simulink model "gofa_robot"  (R2023a)
settings: Solver=FixedStepAuto  StartTime=0.0  StopTime=11  FixedStep=0.001  RelTol=1e-3
undefined symbols (not defined in the file or in its folder): X, Y, Z
libraries: sm_lib x58, nesl_utility x10, slpidlib x3
(part 6 of 7)

== matlab function gofa_robot/gofa_FK2 ==
  data: x output; q1 input; y output; q2 input; q3 input; q4 input; q5 input; q6 input; z output; R output
function [x,y,z,R] = fcn(q1,q2,q3,q4,q5,q6)

R=zeros(3,3);

R(1,1)= (24678615572571482867467662723121*cos(q6)*(cos(q5)*(cos(q3)*(cos(q1)*sin(q2 + pi/2) + (4967757600021511*cos(q2 + pi/2)*sin(q1))/81129638414606681695789005144064) - (4967757600021511*sin(q1))/81129638414606681695789005144064 + sin(q3)*(cos(q1)*cos(q2 + pi/2) - (4967757600021511*sin(q1)*sin(q2 + pi/2))/81129638414606681695789005144064)) + (4967757600021511*cos(q5)*(cos(q4)*sin(q1) + (4967757600021511*cos(q4)*(cos(q3)*(cos(q1)*sin(q2 + pi/2) + (4967757600021511*cos(q2 + pi/2)*sin(q1))/81129638414606681695789005144064) + sin(q3)*(cos(q1)*cos(q2 + pi/2) - (4967757600021511*sin(q1)*sin(q2 + pi/2))/81129638414606681695789005144064)))/81129638414606681695789005144064 + sin(q4)*(cos(q3)*(cos(q1)*cos(q2 + pi/2) - (4967757600021511*sin(q1)*sin(q2 + pi/2))/81129638414606681695789005144064) - sin(q3)*(cos(q1)*sin(q2 + pi/2) + (4967757600021511*cos(q2 + pi/2)*sin(q1))/81129638414606681695789005144064))))/81129638414606681695789005144064 - sin(q5)*(sin(q1)*sin(q4) - cos(q4)*(cos(q3)*(cos(q1)*cos(q2 + pi/2) - (4967757600021511*sin(q1)*sin(q2 + pi/2))/81129638414606681695789005144064) - sin(q3)*(cos(q1)*sin(q2 + pi/2) + (4967757600021511*cos(q2 + pi/2)*sin(q1))/81129638414606681695789005144064)) + (4967757600021511*sin(q4)*(cos(q3)*(cos(q1)*sin(q2 + pi/2) + (4967757600021511*cos(q2 + pi/2)*sin(q1))/81129638414606681695789005144064) + sin(q3)*(cos(q1)*cos(q2 + pi/2) - (4967757600021511*sin(q1)*sin(q2 + pi/2))/81129638414606681695789005144064)))/81129638414606681695789005144064)))/3291009114642412084309938365114701009965471731267159726697218048 - cos(q6)*(sin(q5)*(cos(q3)*(cos(q1)*sin(q2 + pi/2) + (4967757600021511*cos(q2 + pi/2)*sin(q1))/81129638414606681695789005144064) - (4967757600021511*sin(q1))/81129638414606681695789005144064 + sin(q3)*(cos(q1)*cos(q2 + pi/2) - (4967757600021511*sin(q1)*sin(q2 + pi/2))/81129638414606681695789005144064)) + (4967757600021511*sin(q5)*(cos(q4)*sin(q1) + (4967757600021511*cos(q4)*(cos(q3)*(cos(q1)*sin(q2 + pi/2) + (4967757600021511*cos(q2 + pi/2)*sin(q1))/81129638414606681695789005144064) + sin(q3)*(cos(q1)*cos(q2 + pi/2) - (4967757600021511*sin(q1)*sin(q2 + pi/2))/81129638414606681695789005144064)))/81129638414606681695789005144064 + sin(q4)*(cos(q3)*(cos(q1)*cos(q2 + pi/2) - (4967757600021511*sin(q1)*sin(q2 + pi/2))/81129638414606681695789005144064) - sin(q3)*(cos(q1)*sin(q2 + pi/2) + (4967757600021511*cos(q2 + pi/2)*sin(q1))/81129638414606681695789005144064))))/81129638414606681695789005144064 + cos(q5)*(sin(q1)*sin(q4) - cos(q4)*(cos(q3)*(cos(q1)*cos(q2 + pi/2) - (4967757600021511*sin(q1)*sin(q2 + pi/2))/81129638414606681695789005144064) - sin(q3)*(cos(q1)*sin(q2 + pi/2) + (4967757600021511*cos(q2 + pi/2)*sin(q1))/81129638414606681695789005144064)) + (4967757600021511*sin(q4)*(cos(q3)*(cos(q1)*sin(q2 + pi/2) + (4967757600021511*cos(q2 + pi/2)*sin(q1))/81129638414606681695789005144064) + sin(q3)*(cos(q1)*cos(q2 + pi/2) - (4967757600021511*sin(q1)*sin(q2 + pi/2))/81129638414606681695789005144064)))/81129638414606681695789005144064)) - (4967757600021511*sin(q6)*(cos(q5)*(cos(q3)*(cos(q1)*sin(q2 + pi/2) + (4967757600021511*cos(q2 + pi/2)*sin(q1))/81129638414606681695789005144064) - (4967757600021511*sin(q1))/81129638414606681695789005144064 + sin(q3)*(cos(q1)*cos(q2 + pi/2) - (4967757600021511*sin(q1)*sin(q2 + pi/2))/81129638414606681695789005144064)) + (4967757600021511*cos(q5)*(cos(q4)*sin(q1) + (4967757600021511*cos(q4)*(cos(q3)*(cos(q1)*sin(q2 + pi/2) + (4967757600021511*cos(q2 + pi/2)*sin(q1))/81129638414606681695789005144064) + sin(q3)*(cos(q1)*cos(q2 + pi/2) - (4967757600021511*sin(q1)*sin(q2 + pi/2))/81129638414606681695789005144064)))/81129638414606681695789005144064 + sin(q4)*(cos(q3)*(cos(q1)*cos(q2 + pi/2) - (4967757600021511*sin(q1)*sin(q2 + pi/2))/81129638414606681695789005144064) - sin(q3)*(cos(q1)*sin(q2 + pi/2) + (4967757600021511*cos(q2 + pi/2)*sin(q1))/81129638414606681695789005144064))))/81129638414606681695789005144064 - sin(q5)*(sin(q1)*sin(q4) - cos(q4)*(cos(q3)*(cos(q1)*cos(q2 + pi/2) - (4967757600021511*sin(q1)*sin(q2 + pi/2))/81129638414606681695789005144064) - sin(q3)*(cos(q1)*sin(q2 + pi/2) + (4967757600021511*cos(q2 + pi/2)*sin(q1))/81129638414606681695789005144064)) + (4967757600021511*sin(q4)*(cos(q3)*(cos(q1)*sin(q2 + pi/2) + (4967757600021511*cos(q2 + pi/2)*sin(q1))/81129638414606681695789005144064) + sin(q3)*(cos(q1)*cos(q2 + pi/2) - (4967757600021511*sin(q1)*sin(q2 + pi/2))/81129638414606681695789005144064)))/81129638414606681695789005144064)))/81129638414606681695789005144064 - (4967757600021511*sin(q6)*(sin(q5)*(cos(q3)*(cos(q1)*sin(q2 + pi/2) + (4967757600021511*cos(q2 + pi/2)*sin(q1))/81129638414606681695789005144064) - (4967757600021511*sin(q1))/81129638414606681695789005144064 + sin(q3)*(cos(q1)*cos(q2 + pi/2) - (4967757600021511*sin(q1)*sin(q2 + pi/2))/81129638414606681695789005144064)) + (4967757600021511*sin(q5)*(cos(q4)*sin(q1) + (4967757600021511*cos(q4)*(cos(q3)*(cos(q1)*sin(q2 + pi/2) + (4967757600021511*cos(q2 + pi/2)*sin(q1))/81129638414606681695789005144064) + sin(q3)*(cos(q1)*cos(q2 + pi/2) - (4967757600021511*sin(q1)*sin(q2 + pi/2))/81129638414606681695789005144064)))/81129638414606681695789005144064 + sin(q4)*(cos(q3)*(cos(q1)*cos(q2 + pi/2) - (4967757600021511*sin(q1)*sin(q2 + pi/2))/81129638414606681695789005144064) - sin(q3)*(cos(q1)*sin(q2 + pi/2) + (4967757600021511*cos(q2 + pi/2)*sin(q1))/81129638414606681695789005144064))))/81129638414606681695789005144064 + cos(q5)*(sin(q1)*sin(q4) - cos(q4)*(cos(q3)*(cos(q1)*cos(q2 + pi/2) - (4967757600021511*sin(q1)*sin(q2 + pi/2))/81129638414606681695789005144064) - sin(q3)*(cos(q1)*sin(q2 + pi/2) + (4967757600021511*cos(q2 + pi/2)*sin(q1))/81129638414606681695789005144064)) + (4967757600021511*sin(q4)*(cos(q3)*(cos(q1)*sin(q2 + pi/2) + (4967757600021511*cos(q2 + pi/2)*sin(q1))/81129638414606681695789005144064) + sin(q3)*(cos(q1)*cos(q2 + pi/2) - (4967757600021511*sin(q1)*sin(q2 + pi/2))/81129638414606681695789005144064)))/81129638414606681695789005144064)))/40564819207303340847894502572032 + (4967757600021511*cos(q6)*((24678615572571482867467662723121*sin(q1))/6582018229284824168619876730229402019930943462534319453394436096 - (4967757600021511*cos(q3)*(cos(q1)*sin(q2 + pi/2) + (4967757600021511*cos(q2 + pi/2)*sin(q1))/81129638414606681695789005144064))/81129638414606681695789005144064 + cos(q4)*sin(q1) - (4967757600021511*sin(q3)*(cos(q1)*cos(q2 + pi/2) - (4967757600021511*sin(q1)*sin(q2 + pi/2))/81129638414606681695789005144064))/81129638414606681695789005144064 + (4967757600021511*cos(q4)*(cos(q3)*(cos(q1)*sin(q2 + pi/2) + (4967757600021511*cos(q2 + pi/2)*sin(q1))/81129638414606681695789005144064) + sin(q3)*(cos(q1)*cos(q2 + pi/2) - (4967757600021511*sin(q1)*sin(q2 + pi/2))/81129638414606681695789005144064)))/81129638414606681695789005144064 + sin(q4)*(cos(q3)*(cos(q1)*cos(q2 + pi/2) - (4967757600021511*sin(q1)*sin(q2 + pi/2))/81129638414606681695789005144064) - sin(q3)*(cos(q1)*sin(q2 + pi/2) + (4967757600021511*cos(q2 + pi/2)*sin(q1))/81129638414606681695789005144064))))/40564819207303340847894502572032 - sin(q6)*((24678615572571482867467662723121*sin(q1))/6582018229284824168619876730229402019930943462534319453394436096 - (4967757600021511*cos(q3)*(cos(q1)*sin(q2 + pi/2) + (4967757600021511*cos(q2 + pi/2)*sin(q1))/81129638414606681695789005144064))/81129638414606681695789005144064 + cos(q4)*sin(q1) - (4967757600021511*sin(q3)*(cos(q1)*cos(q2 + pi/2) - (4967757600021511*sin(q1)*sin(q2 + pi/2))/81129638414606681695789005144064))/81129638414606681695789005144064 + (4967757600021511*cos(q4)*(cos(q3)*(cos(q1)*sin(q2 + pi/2) + (4967757600021511*cos(q2 + pi/2)*sin(q1))/81129638414606681695789005144064) + sin(q3)*(cos(q1)*cos(q2 + pi/2) - (4967757600021511*sin(q1)*sin(q2 + pi/2))/81129638414606681695789005144064)))/81129638414606681695789005144064 + sin(q4)*(cos(q3)*(cos(q1)*cos(q2 + pi/2) - (4967757600021511*sin(q1)*sin(q2 + pi/2))/81129638414606681695789005144064) - sin(q3)*(cos(q1)*sin(q2 + pi/2) + (4967757600021511*cos(q2 + pi/2)*sin(q1))/81129638414606681695789005144064)));
R(1,2)= sin(q6)*(sin(q5)*(cos(q3)*(cos(q1)*sin(q2 + pi/2) + (4967757600021511*cos(q2 + pi/2)*sin(q1))/81129638414606681695789005144064) - (4967757600021511*sin(q1))/81129638414606681695789005144064 + sin(q3)*(cos(q1)*cos(q2 + pi/2) - (4967757600021511*sin(q1)*sin(q2 + pi/2))/81129638414606681695789005144064)) + (4967757600021511*sin(q5)*(cos(q4)*sin(q1) + (4967757600021511*cos(q4)*(cos(q3)*(cos(q1)*sin(q2 + pi/2) + (4967757600021511*cos(q2 + pi/2)*sin(q1))/81129638414606681695789005144064) + sin(q3)*(cos(q1)*cos(q2 + pi/2) - (4967757600021511*sin(q1)*sin(q2 + pi/2))/81129638414606681695789005144064)))/81129638414606681695789005144064 + sin(q4)*(cos(q3)*(cos(q1)*cos(q2 + pi/2) - (4967757600021511*sin(q1)*sin(q2 + pi/2))/81129638414606681695789005144064) - sin(q3)*(cos(q1)*sin(q2 + pi/2) + (4967757600021511*cos(q2 + pi/2)*sin(q1))/81129638414606681695789005144064))))/81129638414606681695789005144064 + cos(q5)*(sin(q1)*sin(q4) - cos(q4)*(cos(q3)*(cos(q1)*cos(q2 + pi/2) - (4967757600021511*sin(q1)*sin(q2 + pi/2))/81129638414606681695789005144064) - sin(q3)*(cos(q1)*sin(q2 + pi/2) + (4967757600021511*cos(q2 + pi/2)*sin(q1))/81129638414606681695789005144064)) + (4967757600021511*sin(q4)*(cos(q3)*(cos(q1)*sin(q2 + pi/2) + (4967757600021511*cos(q2 + pi/2)*sin(q1))/81129638414606681695789005144064) + sin(q3)*(cos(q1)*cos(q2 + pi/2) - (4967757600021511*sin(q1)*sin(q2 + pi/2))/81129638414606681695789005144064)))/81129638414606681695789005144064)) - (4967757600021511*cos(q6)*(sin(q5)*(cos(q3)*(cos(q1)*sin(q2 + pi/2) + (4967757600021511*cos(q2 + pi/2)*sin(q1))/81129638414606681695789005144064) - (4967757600021511*sin(q1))/81129638414606681695789005144064 + sin(q3)*(cos(q1)*cos(q2 + pi/2) - (4967757600021511*sin(q1)*sin(q2 + pi/2))/81129638414606681695789005144064)) + (4967757600021511*sin(q5)*(cos(q4)*sin(q1) + (4967757600021511*cos(q4)*(cos(q3)*(cos(q1)*sin(q2 + pi/2) + (4967757600021511*cos(q2 + pi/2)*sin(q1))/81129638414606681695789005144064) + sin(q3)*(cos(q1)*cos(q2 + pi/2) - (4967757600021511*sin(q1)*sin(q2 + pi/2))/81129638414606681695789005144064)))/81129638414606681695789005144064 + sin(q4)*(cos(q3)*(cos(q1)*cos(q2 + pi/2) - (4967757600021511*sin(q1)*sin(q2 + pi/2))/81129638414606681695789005144064) - sin(q3)*(cos(q1)*sin(q2 + pi/2) + (4967757600021511*cos(q2 + pi/2)*sin(q1))/81129638414606681695789005144064))))/81129638414606681695789005144064 + cos(q5)*(sin(q1)*sin(q4) - cos(q4)*(cos(q3)*(cos(q1)*cos(q2 + pi/2) - (4967757600021511*sin(q1)*sin(q2 + pi/2))/81129638414606681695789005144064) - sin(q3)*(cos(q1)*sin(q2 + pi/2) + (4967757600021511*cos(q2 + pi/2)*sin(q1))/81129638414606681695789005144064)) + (4967757600021511*sin(q4)*(cos(q3)*(cos(q1)*sin(q2 + pi/2) + (4967757600021511*cos(q2 + pi/2)*sin(q1))/81129638414606681695789005144064) + sin(q3)*(cos(q1)*cos(q2 + pi/2) - (4967757600021511*sin(q1)*sin(q2 + pi/2))/81129638414606681695789005144064)))/81129638414606681695789005144064)))/40564819207303340847894502572032 - (24678615572571482867467662723121*sin(q6)*(cos(q5)*(cos(q3)*(cos(q1)*sin(q2 + pi/2) + (4967757600021511*cos(q2 + pi/2)*sin(q1))/81129638414606681695789005144064) - (4967757600021511*sin(q1))/81129638414606681695789005144064 + sin(q3)*(cos(q1)*cos(q2 + pi/2) - (4967757600021511*sin(q1)*sin(q2 + pi/2))/81129638414606681695789005144064)) + (4967757600021511*cos(q5)*(cos(q4)*sin(q1) + (4967757600021511*cos(q4)*(cos(q3)*(cos(q1)*sin(q2 + pi/2) + (4967757600021511*cos(q2 + pi/2)*sin(q1))/81129638414606681695789005144064) + sin(q3)*(cos(q1)*cos(q2 + pi/2) - (4967757600021511*sin(q1)*sin(q2 + pi/2))/81129638414606681695789005144064)))/81129638414606681695789005144064 + sin(q4)*(cos(q3)*(cos(q1)*cos(q2 + pi/2) - (4967757600021511*sin(q1)*sin(q2 + pi/2))/81129638414606681695789005144064) - sin(q3)*(cos(q1)*sin(q2 + pi/2) + (4967757600021511*cos(q2 + pi/2)*sin(q1))/81129638414606681695789005144064))))/81129638414606681695789005144064 - sin(q5)*(sin(q1)*sin(q4) - cos(q4)*(cos(q3)*(cos(q1)*cos(q2 + pi/2) - (4967757600021511*sin(q1)*sin(q2 + pi/2))/81129638414606681695789005144064) - sin(q3)*(cos(q1)*sin(q2 + pi/2) + (4967757600021511*cos(q2 + pi/2)*sin(q1))/81129638414606681695789005144064)) + (4967757600021511*sin(q4)*(cos(q3)*(cos(q1)*sin(q2 + pi/2) + (4967757600021511*cos(q2 + pi/2)*sin(q1))/81129638414606681695789005144064) + sin(q3)*(cos(q1)*cos(q2 + pi/2) - (4967757600021511*sin(q1)*sin(q2 + pi/2))/81129638414606681695789005144064)))/81129638414606681695789005144064)))/3291009114642412084309938365114701009965471731267159726697218048 - (4967757600021511*cos(q6)*(cos(q5)*(cos(q3)*(cos(q1)*sin(q2 + pi/2) + (4967757600021511*cos(q2 + pi/2)*sin(q1))/81129638414606681695789005144064) - (4967757600021511*sin(q1))/81129638414606681695789005144064 + sin(q3)*(cos(q1)*cos(q2 + pi/2) - (4967757600021511*sin(q1)*sin(q2 + pi/2))/81129638414606681695789005144064)) + (4967757600021511*cos(q5)*(cos(q4)*sin(q1) + (4967757600021511*cos(q4)*(cos(q3)*(cos(q1)*sin(q2 + pi/2) + (4967757600021511*cos(q2 + pi/2)*sin(q1))/81129638414606681695789005144064) + sin(q3)*(cos(q1)*cos(q2 + pi/2) - (4967757600021511*sin(q1)*sin(q2 + pi/2))/81129638414606681695789005144064)))/81129638414606681695789005144064 + sin(q4)*(cos(q3)*(cos(q1)*cos(q2 + pi/2) - (4967757600021511*sin(q1)*sin(q2 + pi/2))/81129638414606681695789005144064) - sin(q3)*(cos(q1)*sin(q2 + pi/2) + (4967757600021511*cos(q2 + pi/2)*sin(q1))/81129638414606681695789005144064))))/81129638414606681695789005144064 - sin(q5)*(sin(q1)*sin(q4) - cos(q4)*(cos(q3)*(cos(q1)*cos(q2 + pi/2) - (4967757600021511*sin(q1)*sin(q2 + pi/2))/81129638414606681695789005144064) - sin(q3)*(cos(q1)*sin(q2 + pi/2) + (4967757600021511*cos(q2 + pi/2)*sin(q1))/81129638414606681695789005144064)) + (4967757600021511*sin(q4)*(cos(q3)*(cos(q1)*sin(q2 + pi/2) + (4967757600021511*cos(q2 + pi/2)*sin(q1))/81129638414606681695789005144064) + sin(q3)*(cos(q1)*cos(q2 + pi/2) - (4967757600021511*sin(q1)*sin(q2 + pi/2))/81129638414606681695789005144064)))/81129638414606681695789005144064)))/81129638414606681695789005144064 - cos(q6)*((24678615572571482867467662723121*sin(q1))/6582018229284824168619876730229402019930943462534319453394436096 - (4967757600021511*cos(q3)*(cos(q1)*sin(q2 + pi/2) + (4967757600021511*cos(q2 + pi/2)*sin(q1))/81129638414606681695789005144064))/81129638414606681695789005144064 + cos(q4)*sin(q1) - (4967757600021511*sin(q3)*(cos(q1)*cos(q2 + pi/2) - (4967757600021511*sin(q1)*sin(q2 + pi/2))/81129638414606681695789005144064))/81129638414606681695789005144064 + (4967757600021511*cos(q4)*(cos(q3)*(cos(q1)*sin(q2 + pi/2) + (4967757600021511*cos(q2 + pi/2)*sin(q1))/81129638414606681695789005144064) + sin(q3)*(cos(q1)*cos(q2 + pi/2) - (4967757600021511*sin(q1)*sin(q2 + pi/2))/81129638414606681695789005144064)))/81129638414606681695789005144064 + sin(q4)*(cos(q3)*(cos(q1)*cos(q2 + pi/2) - (4967757600021511*sin(q1)*sin(q2 + pi/2))/81129638414606681695789005144064) - sin(q3)*(cos(q1)*sin(q2 + pi/2) + (4967757600021511*cos(q2 + pi/2)*sin(q1))/81129638414606681695789005144064))) - (4967757600021511*sin(q6)*((24678615572571482867467662723121*sin(q1))/6582018229284824168619876730229402019930943462534319453394436096 - (4967757600021511*cos(q3)*(cos(q1)*sin(q2 + pi/2) + (4967757600021511*cos(q2 + pi/2)*sin(q1))/81129638414606681695789005144064))/81129638414606681695789005144064 + cos(q4)*sin(q1) - (4967757600021511*sin(q3)*(cos(q1)*cos(q2 + pi/2) - (4967757600021511*sin(q1)*sin(q2 + pi/2))/81129638414606681695789005144064))/81129638414606681695789005144064 + (4967757600021511*cos(q4)*(cos(q3)*(cos(q1)*sin(q2 + pi/2) + (4967757600021511*cos(q2 + pi/2)*sin(q1))/81129638414606681695789005144064) + sin(q3)*(cos(q1)*cos(q2 + pi/2) - (4967757600021511*sin(q1)*sin(q2 + pi/2))/81129638414606681695789005144064)))/81129638414606681695789005144064 + sin(q4)*(cos(q3)*(cos(q1)*cos(q2 + pi/2) - (4967757600021511*sin(q1)*sin(q2 + pi/2))/81129638414606681695789005144064) - sin(q3)*(cos(q1)*sin(q2 + pi/2) + (4967757600021511*cos(q2 + pi/2)*sin(q1))/81129638414606681695789005144064))))/40564819207303340847894502572032; 
R(1,3)= (24678615572571482867467662723121*cos(q3)*(cos(q1)*sin(q2 + pi/2) + (4967757600021511*cos(q2 + pi/2)*sin(q1))/81129638414606681695789005144064))/6582018229284824168619876730229402019930943462534319453394436096 - (122597380068651197257713859414983140362437055831*sin(q1))/533996758980227520598755426542388028650676130589163192486760401955554931445160137505740521734144 - (4967757600021511*cos(q4)*sin(q1))/81129638414606681695789005144064 + (24678615572571482867467662723121*sin(q3)*(cos(q1)*cos(q2 + pi/2) - (4967757600021511*sin(q1)*sin(q2 + pi/2))/81129638414606681695789005144064))/6582018229284824168619876730229402019930943462534319453394436096 + cos(q5)*(cos(q3)*(cos(q1)*sin(q2 + pi/2) + (4967757600021511*cos(q2 + pi/2)*sin(q1))/81129638414606681695789005144064) - (4967757600021511*sin(q1))/81129638414606681695789005144064 + sin(q3)*(cos(q1)*cos(q2 + pi/2) - (4967757600021511*sin(q1)*sin(q2 + pi/2))/81129638414606681695789005144064)) + (4967757600021511*cos(q5)*(cos(q4)*sin(q1) + (4967757600021511*cos(q4)*(cos(q3)*(cos(q1)*sin(q2 + pi/2) + (4967757600021511*cos(q2 + pi/2)*sin(q1))/81129638414606681695789005144064) + sin(q3)*(cos(q1)*cos(q2 + pi/2) - (4967757600021511*sin(q1)*sin(q2 + pi/2))/81129638414606681695789005144064)))/81129638414606681695789005144064 + sin(q4)*(cos(q3)*(cos(q1)*cos(q2 + pi/2) - (4967757600021511*sin(q1)*sin(q2 + pi/2))/81129638414606681695789005144064) - sin(q3)*(cos(q1)*sin(q2 + pi/2) + (4967757600021511*cos(q2 + pi/2)*sin(q1))/81129638414606681695789005144064))))/81129638414606681695789005144064 - sin(q5)*(sin(q1)*sin(q4) - cos(q4)*(cos(q3)*(cos(q1)*cos(q2 + pi/2) - (4967757600021511*sin(q1)*sin(q2 + pi/2))/81129638414606681695789005144064) - sin(q3)*(cos(q1)*sin(q2 + pi/2) + (4967757600021511*cos(q2 + pi/2)*sin(q1))/81129638414606681695789005144064)) + (4967757600021511*sin(q4)*(cos(q3)*(cos(q1)*sin(q2 + pi/2) + (4967757600021511*cos(q2 + pi/2)*sin(q1))/81129638414606681695789005144064) + sin(q3)*(cos(q1)*cos(q2 + pi/2) - (4967757600021511*sin(q1)*sin(q2 + pi/2))/81129638414606681695789005144064)))/81129638414606681695789005144064) - (24678615572571482867467662723121*cos(q4)*(cos(q3)*(cos(q1)*sin(q2 + pi/2) + (4967757600021511*cos(q2 + pi/2)*sin(q1))/81129638414606681695789005144064) + sin(q3)*(cos(q1)*cos(q2 + pi/2) - (4967757600021511*sin(q1)*sin(q2 + pi/2))/81129638414606681695789005144064)))/6582018229284824168619876730229402019930943462534319453394436096 - (4967757600021511*sin(q4)*(cos(q3)*(cos(q1)*cos(q2 + pi/2) - (4967757600021511*sin(q1)*sin(q2 + pi/2))/81129638414606681695789005144064) - sin(q3)*(cos(q1)*sin(q2 + pi/2) + (4967757600021511*cos(q2 + pi/2)*sin(q1))/81129638414606681695789005144064)))/81129638414606681695789005144064;
R(2,1)= (24678615572571482867467662723121*cos(q6)*(cos(q5)*((4967757600021511*cos(q1))/81129638414606681695789005144064 - cos(q3)*((4967757600021511*cos(q1)*cos(q2 + pi/2))/81129638414606681695789005144064 - sin(q1)*sin(q2 + pi/2)) + sin(q3)*((4967757600021511*cos(q1)*sin(q2 + pi/2))/81129638414606681695789005144064 + cos(q2 + pi/2)*sin(q1))) - (4967757600021511*cos(q5)*(cos(q1)*cos(q4) + (4967757600021511*cos(q4)*(cos(q3)*((4967757600021511*cos(q1)*cos(q2 + pi/2))/81129638414606681695789005144064 - sin(q1)*sin(q2 + pi/2)) - sin(q3)*((4967757600021511*cos(q1)*sin(q2 + pi/2))/81129638414606681695789005144064 + cos(q2 + pi/2)*sin(q1))))/81129638414606681695789005144064 - sin(q4)*(cos(q3)*((4967757600021511*cos(q1)*sin(q2 + pi/2))/81129638414606681695789005144064 + cos(q2 + pi/2)*sin(q1)) + sin(q3)*((4967757600021511*cos(q1)*cos(q2 + pi/2))/81129638414606681695789005144064 - sin(q1)*sin(q2 + pi/2)))))/81129638414606681695789005144064 + sin(q5)*(cos(q1)*sin(q4) + cos(q4)*(cos(q3)*((4967757600021511*cos(q1)*sin(q2 + pi/2))/81129638414606681695789005144064 + cos(q2 + pi/2)*sin(q1)) + sin(q3)*((4967757600021511*cos(q1)*cos(q2 + pi/2))/81129638414606681695789005144064 - sin(q1)*sin(q2 + pi/2))) + (4967757600021511*sin(q4)*(cos(q3)*((4967757600021511*cos(q1)*cos(q2 + pi/2))/81129638414606681695789005144064 - sin(q1)*sin(q2 + pi/2)) - sin(q3)*((4967757600021511*cos(q1)*sin(q2 + pi/2))/81129638414606681695789005144064 + cos(q2 + pi/2)*sin(q1))))/81129638414606681695789005144064)))/3291009114642412084309938365114701009965471731267159726697218048 - (4967757600021511*sin(q6)*(cos(q5)*((4967757600021511*cos(q1))/81129638414606681695789005144064 - cos(q3)*((4967757600021511*cos(q1)*cos(q2 + pi/2))/81129638414606681695789005144064 - sin(q1)*sin(q2 + pi/2)) + sin(q3)*((4967757600021511*cos(q1)*sin(q2 + pi/2))/81129638414606681695789005144064 + cos(q2 + pi/2)*sin(q1))) - (4967757600021511*cos(q5)*(cos(q1)*cos(q4) + (4967757600021511*cos(q4)*(cos(q3)*((4967757600021511*cos(q1)*cos(q2 + pi/2))/81129638414606681695789005144064 - sin(q1)*sin(q2 + pi/2)) - sin(q3)*((4967757600021511*cos(q1)*sin(q2 + pi/2))/81129638414606681695789005144064 + cos(q2 + pi/2)*sin(q1))))/81129638414606681695789005144064 - sin(q4)*(cos(q3)*((4967757600021511*cos(q1)*sin(q2 + pi/2))/81129638414606681695789005144064 + cos(q2 + pi/2)*sin(q1)) + sin(q3)*((4967757600021511*cos(q1)*cos(q2 + pi/2))/81129638414606681695789005144064 - sin(q1)*sin(q2 + pi/2)))))/81129638414606681695789005144064 + sin(q5)*(cos(q1)*sin(q4) + cos(q4)*(cos(q3)*((4967757600021511*cos(q1)*sin(q2 + pi/2))/81129638414606681695789005144064 + cos(q2 + pi/2)*sin(q1)) + sin(q3)*((4967757600021511*cos(q1)*cos(q2 + pi/2))/81129638414606681695789005144064 - sin(q1)*sin(q2 + pi/2))) + (4967757600021511*sin(q4)*(cos(q3)*((4967757600021511*cos(q1)*cos(q2 + pi/2))/81129638414606681695789005144064 - sin(q1)*sin(q2 + pi/2)) - sin(q3)*((4967757600021511*cos(q1)*sin(q2 + pi/2))/81129638414606681695789005144064 + cos(q2 + pi/2)*sin(q1))))/81129638414606681695789005144064)))/81129638414606681695789005144064 + cos(q6)*(cos(q5)*(cos(q1)*sin(q4) + cos(q4)*(cos(q3)*((4967757600021511*cos(q1)*sin(q2 + pi/2))/81129638414606681695789005144064 + cos(q2 + pi/2)*sin(q1)) + sin(q3)*((4967757600021511*cos(q1)*cos(q2 + pi/2))/81129638414606681695789005144064 - sin(q1)*sin(q2 + pi/2))) + (4967757600021511*sin(q4)*(cos(q3)*((4967757600021511*cos(q1)*cos(q2 + pi/2))/81129638414606681695789005144064 - sin(q1)*sin(q2 + pi/2)) - sin(q3)*((4967757600021511*cos(q1)*sin(q2 + pi/2))/81129638414606681695789005144064 + cos(q2 + pi/2)*sin(q1))))/81129638414606681695789005144064) - sin(q5)*((4967757600021511*cos(q1))/81129638414606681695789005144064 - cos(q3)*((4967757600021511*cos(q1)*cos(q2 + pi/2))/81129638414606681695789005144064 - sin(q1)*sin(q2 + pi/2)) + sin(q3)*((4967757600021511*cos(q1)*sin(q2 + pi/2))/81129638414606681695789005144064 + cos(q2 + pi/2)*sin(q1))) + (4967757600021511*sin(q5)*(cos(q1)*cos(q4) + (4967757600021511*cos(q4)*(cos(q3)*((4967757600021511*cos(q1)*cos(q2 + pi/2))/81129638414606681695789005144064 - sin(q1)*sin(q2 + pi/2)) - sin(q3)*((4967757600021511*cos(q1)*sin(q2 + pi/2))/81129638414606681695789005144064 + cos(q2 + pi/2)*sin(q1))))/81129638414606681695789005144064 - sin(q4)*(cos(q3)*((4967757600021511*cos(q1)*sin(q2 + pi/2))/81129638414606681695789005144064 + cos(q2 + pi/2)*sin(q1)) + sin(q3)*((4967757600021511*cos(q1)*cos(q2 + pi/2))/81129638414606681695789005144064 - sin(q1)*sin(q2 + pi/2)))))/81129638414606681695789005144064) + (4967757600021511*sin(q6)*(cos(q5)*(cos(q1)*sin(q4) + cos(q4)*(cos(q3)*((4967757600021511*cos(q1)*sin(q2 + pi/2))/81129638414606681695789005144064 + cos(q2 + pi/2)*sin(q1)) + sin(q3)*((4967757600021511*cos(q1)*cos(q2 + pi/2))/81129638414606681695789005144064 - sin(q1)*sin(q2 + pi/2))) + (4967757600021511*sin(q4)*(cos(q3)*((4967757600021511*cos(q1)*cos(q2 + pi/2))/81129638414606681695789005144064 - sin(q1)*sin(q2 + pi/2)) - sin(q3)*((4967757600021511*cos(q1)*sin(q2 + pi/2))/81129638414606681695789005144064 + cos(q2 + pi/2)*sin(q1))))/81129638414606681695789005144064) - sin(q5)*((4967757600021511*cos(q1))/81129638414606681695789005144064 - cos(q3)*((4967757600021511*cos(q1)*cos(q2 + pi/2))/81129638414606681695789005144064 - sin(q1)*sin(q2 + pi/2)) + sin(q3)*((4967757600021511*cos(q1)*sin(q2 + pi/2))/81129638414606681695789005144064 + cos(q2 + pi/2)*sin(q1))) + (4967757600021511*sin(q5)*(cos(q1)*cos(q4) + (4967757600021511*cos(q4)*(cos(q3)*((4967757600021511*cos(q1)*cos(q2 + pi/2))/81129638414606681695789005144064 - sin(q1)*sin(q2 + pi/2)) - sin(q3)*((4967757600021511*cos(q1)*sin(q2 + pi/2))/81129638414606681695789005144064 + cos(q2 + pi/2)*sin(q1))))/81129638414606681695789005144064 - sin(q4)*(cos(q3)*((4967757600021511*cos(q1)*sin(q2 + pi/2))/81129638414606681695789005144064 + cos(q2 + pi/2)*sin(q1)) + sin(q3)*((4967757600021511*cos(q1)*cos(q2 + pi/2))/81129638414606681695789005144064 - sin(q1)*sin(q2 + pi/2)))))/81129638414606681695789005144064))/40564819207303340847894502572032 - (4967757600021511*cos(q6)*((24678615572571482867467662723121*cos(q1))/6582018229284824168619876730229402019930943462534319453394436096 + cos(q1)*cos(q4) - (4967757600021511*cos(q3)*((4967757600021511*cos(q1)*cos(q2 + pi/2))/81129638414606681695789005144064 - sin(q1)*sin(q2 + pi/2)))/81129638414606681695789005144064 + (4967757600021511*sin(q3)*((4967757600021511*cos(q1)*sin(q2 + pi/2))/81129638414606681695789005144064 + cos(q2 + pi/2)*sin(q1)))/81129638414606681695789005144064 + (4967757600021511*cos(q4)*(cos(q3)*((4967757600021511*cos(q1)*cos(q2 + pi/2))/81129638414606681695789005144064 - sin(q1)*sin(q2 + pi/2)) - sin(q3)*((4967757600021511*cos(q1)*sin(q2 + pi/2))/81129638414606681695789005144064 + cos(q2 + pi/2)*sin(q1))))/81129638414606681695789005144064 - sin(q4)*(cos(q3)*((4967757600021511*cos(q1)*sin(q2 + pi/2))/81129638414606681695789005144064 + cos(q2 + pi/2)*sin(q1)) + sin(q3)*((4967757600021511*cos(q1)*cos(q2 + pi/2))/81129638414606681695789005144064 - sin(q1)*sin(q2 + pi/2)))))/40564819207303340847894502572032 + sin(q6)*((24678615572571482867467662723121*cos(q1))/6582018229284824168619876730229402019930943462534319453394436096 + cos(q1)*cos(q4) - (4967757600021511*cos(q3)*((4967757600021511*cos(q1)*cos(q2 + pi/2))/81129638414606681695789005144064 - sin(q1)*sin(q2 + pi/2)))/81129638414606681695789005144064 + (4967757600021511*sin(q3)*((4967757600021511*cos(q1)*sin(q2 + pi/2))/81129638414606681695789005144064 + cos(q2 + pi/2)*sin(q1)))/81129638414606681695789005144064 + (4967757600021511*cos(q4)*(cos(q3)*((4967757600021511*cos(q1)*cos(q2 + pi/2))/81129638414606681695789005144064 - sin(q1)*sin(q2 + pi/2)) - sin(q3)*((4967757600021511*cos(q1)*sin(q2 + pi/2))/81129638414606681695789005144064 + cos(q2 + pi/2)*sin(q1))))/81129638414606681695789005144064 - sin(q4)*(cos(q3)*((4967757600021511*cos(q1)*sin(q2 + pi/2))/81129638414606681695789005144064 + cos(q2 + pi/2)*sin(q1)) + sin(q3)*((4967757600021511*cos(q1)*cos(q2 + pi/2))/81129638414606681695789005144064 - sin(q1)*sin(q2 + pi/2)))); 
R(2,2)= (4967757600021511*cos(q6)*(cos(q5)*(cos(q1)*sin(q4) + cos(q4)*(cos(q3)*((4967757600021511*cos(q1)*sin(q2 + pi/2))/81129638414606681695789005144064 + cos(q2 + pi/2)*sin(q1)) + sin(q3)*((4967757600021511*cos(q1)*cos(q2 + pi/2))/81129638414606681695789005144064 - sin(q1)*sin(q2 + pi/2))) + (4967757600021511*sin(q4)*(cos(q3)*((4967757600021511*cos(q1)*cos(q2 + pi/2))/81129638414606681695789005144064 - sin(q1)*sin(q2 + pi/2)) - sin(q3)*((4967757600021511*cos(q1)*sin(q2 + pi/2))/81129638414606681695789005144064 + cos(q2 + pi/2)*sin(q1))))/81129638414606681695789005144064) - sin(q5)*((4967757600021511*cos(q1))/81129638414606681695789005144064 - cos(q3)*((4967757600021511*cos(q1)*cos(q2 + pi/2))/81129638414606681695789005144064 - sin(q1)*sin(q2 + pi/2)) + sin(q3)*((4967757600021511*cos(q1)*sin(q2 + pi/2))/81129638414606681695789005144064 + cos(q2 + pi/2)*sin(q1))) + (4967757600021511*sin(q5)*(cos(q1)*cos(q4) + (4967757600021511*cos(q4)*(cos(q3)*((4967757600021511*cos(q1)*cos(q2 + pi/2))/81129638414606681695789005144064 - sin(q1)*sin(q2 + pi/2)) - sin(q3)*((4967757600021511*cos(q1)*sin(q2 + pi/2))/81129638414606681695789005144064 + cos(q2 + pi/2)*sin(q1))))/81129638414606681695789005144064 - sin(q4)*(cos(q3)*((4967757600021511*cos(q1)*sin(q2 + pi/2))/81129638414606681695789005144064 + cos(q2 + pi/2)*sin(q1)) + sin(q3)*((4967757600021511*cos(q1)*cos(q2 + pi/2))/81129638414606681695789005144064 - sin(q1)*sin(q2 + pi/2)))))/81129638414606681695789005144064))/40564819207303340847894502572032 - (24678615572571482867467662723121*sin(q6)*(cos(q5)*((4967757600021511*cos(q1))/81129638414606681695789005144064 - cos(q3)*((4967757600021511*cos(q1)*cos(q2 + pi/2))/81129638414606681695789005144064 - sin(q1)*sin(q2 + pi/2)) + sin(q3)*((4967757600021511*cos(q1)*sin(q2 + pi/2))/81129638414606681695789005144064 + cos(q2 + pi/2)*sin(q1))) - (4967757600021511*cos(q5)*(cos(q1)*cos(q4) + (4967757600021511*cos(q4)*(cos(q3)*((4967757600021511*cos(q1)*cos(q2 + pi/2))/81129638414606681695789005144064 - sin(q1)*sin(q2 + pi/2)) - sin(q3)*((4967757600021511*cos(q1)*sin(q2 + pi/2))/81129638414606681695789005144064 + cos(q2 + pi/2)*sin(q1))))/81129638414606681695789005144064 - sin(q4)*(cos(q3)*((4967757600021511*cos(q1)*sin(q2 + pi/2))/81129638414606681695789005144064 + cos(q2 + pi/2)*sin(q1)) + sin(q3)*((4967757600021511*cos(q1)*cos(q2 + pi/2))/81129638414606681695789005144064 - sin(q1)*sin(q2 + pi/2)))))/81129638414606681695789005144064 + sin(q5)*(cos(q1)*sin(q4) + cos(q4)*(cos(q3)*((4967757600021511*cos(q1)*sin(q2 + pi/2))/81129638414606681695789005144064 + cos(q2 + pi/2)*sin(q1)) + sin(q3)*((4967757600021511*cos(q1)*cos(q2 + pi/2))/81129638414606681695789005144064 - sin(q1)*sin(q2 + pi/2))) + (4967757600021511*sin(q4)*(cos(q3)*((4967757600021511*cos(q1)*cos(q2 + pi/2))/81129638414606681695789005144064 - sin(q1)*sin(q2 + pi/2)) - sin(q3)*((4967757600021511*cos(q1)*sin(q2 + pi/2))/81129638414606681695789005144064 + cos(q2 + pi/2)*sin(q1))))/81129638414606681695789005144064)))/3291009114642412084309938365114701009965471731267159726697218048 - (4967757600021511*cos(q6)*(cos(q5)*((4967757600021511*cos(q1))/81129638414606681695789005144064 - cos(q3)*((4967757600021511*cos(q1)*cos(q2 + pi/2))/81129638414606681695789005144064 - sin(q1)*sin(q2 + pi/2)) + sin(q3)*((4967757600021511*cos(q1)*sin(q2 + pi/2))/81129638414606681695789005144064 + cos(q2 + pi/2)*sin(q1))) - (4967757600021511*cos(q5)*(cos(q1)*cos(q4) + (4967757600021511*cos(q4)*(cos(q3)*((4967757600021511*cos(q1)*cos(q2 + pi/2))/81129638414606681695789005144064 - sin(q1)*sin(q2 + pi/2)) - sin(q3)*((4967757600021511*cos(q1)*sin(q2 + pi/2))/81129638414606681695789005144064 + cos(q2 + pi/2)*sin(q1))))/81129638414606681695789005144064 - sin(q4)*(cos(q3)*((4967757600021511*cos(q1)*sin(q2 + pi/2))/81129638414606681695789005144064 + cos(q2 + pi/2)*sin(q1)) + sin(q3)*((4967757600021511*cos(q1)*cos(q2 + pi/2))/81129638414606681695789005144064 - sin(q1)*sin(q2 + pi/2)))))/81129638414606681695789005144064 + sin(q5)*(cos(q1)*sin(q4) + cos(q4)*(cos(q3)*((4967757600021511*cos(q1)*sin(q2 + pi/2))/81129638414606681695789005144064 + cos(q2 + pi/2)*sin(q1)) + sin(q3)*((4967757600021511*cos(q1)*cos(q2 + pi/2))/81129638414606681695789005144064 - sin(q1)*sin(q2 + pi/2))) + (4967757600021511*sin(q4)*(cos(q3)*((4967757600021511*cos(q1)*cos(q2 + pi/2))/81129638414606681695789005144064 - sin(q1)*sin(q2 + pi/2)) - sin(q3)*((4967757600021511*cos(q1)*sin(q2 + pi/2))/81129638414606681695789005144064 + cos(q2 + pi/2)*sin(q1))))/81129638414606681695789005144064)))/81129638414606681695789005144064 - sin(q6)*(cos(q5)*(cos(q1)*sin(q4) + cos(q4)*(cos(q3)*((4967757600021511*cos(q1)*sin(q2 + pi/2))/81129638414606681695789005144064 + cos(q2 + pi/2)*sin(q1)) + sin(q3)*((4967757600021511*cos(q1)*cos(q2 + pi/2))/81129638414606681695789005144064 - sin(q1)*sin(q2 + pi/2))) + (4967757600021511*sin(q4)*(cos(q3)*((4967757600021511*cos(q1)*cos(q2 + pi/2))/81129638414606681695789005144064 - sin(q1)*sin(q2 + pi/2)) - sin(q3)*((4967757600021511*cos(q1)*sin(q2 + pi/2))/81129638414606681695789005144064 + cos(q2 + pi/2)*sin(q1))))/81129638414606681695789005144064) - sin(q5)*((4967757600021511*cos(q1))/81129638414606681695789005144064 - cos(q3)*((4967757600021511*cos(q1)*cos(q2 + pi/2))/81129638414606681695789005144064 - sin(q1)*sin(q2 + pi/2)) + sin(q3)*((4967757600021511*cos(q1)*sin(q2 + pi/2))/81129638414606681695789005144064 + cos(q2 + pi/2)*sin(q1))) + (4967757600021511*sin(q5)*(cos(q1)*cos(q4) + (4967757600021511*cos(q4)*(cos(q3)*((4967757600021511*cos(q1)*cos(q2 + pi/2))/81129638414606681695789005144064 - sin(q1)*sin(q2 + pi/2)) - sin(q3)*((4967757600021511*cos(q1)*sin(q2 + pi/2))/81129638414606681695789005144064 + cos(q2 + pi/2)*sin(q1))))/81129638414606681695789005144064 - sin(q4)*(cos(q3)*((4967757600021511*cos(q1)*sin(q2 + pi/2))/81129638414606681695789005144064 + cos(q2 + pi/2)*sin(q1)) + sin(q3)*((4967757600021511*cos(q1)*cos(q2 + pi/2))/81129638414606681695789005144064 - sin(q1)*sin(q2 + pi/2)))))/81129638414606681695789005144064) + cos(q6)*((24678615572571482867467662723121*cos(q1))/6582018229284824168619876730229402019930943462534319453394436096 + cos(q1)*cos(q4) - (4967757600021511*cos(q3)*((4967757600021511*cos(q1)*cos(q2 + pi/2))/81129638414606681695789005144064 - sin(q1)*sin(q2 + pi/2)))/81129638414606681695789005144064 + (4967757600021511*sin(q3)*((4967757600021511*cos(q1)*sin(q2 + pi/2))/81129638414606681695789005144064 + cos(q2 + pi/2)*sin(q1)))/81129638414606681695789005144064 + (4967757600021511*cos(q4)*(cos(q3)*((4967757600021511*cos(q1)*cos(q2 + pi/2))/81129638414606681695789005144064 - sin(q1)*sin(q2 + pi/2)) - sin(q3)*((4967757600021511*cos(q1)*sin(q2 + pi/2))/81129638414606681695789005144064 + cos(q2 + pi/2)*sin(q1))))/81129638414606681695789005144064 - sin(q4)*(cos(q3)*((4967757600021511*cos(q1)*sin(q2 + pi/2))/81129638414606681695789005144064 + cos(q2 + pi/2)*sin(q1)) + sin(q3)*((4967757600021511*cos(q1)*cos(q2 + pi/2))/81129638414606681695789005144064 - sin(q1)*sin(q2 + pi/2)))) + (4967757600021511*sin(q6)*((24678615572571482867467662723121*cos(q1))/6582018229284824168619876730229402019930943462534319453394436096 + cos(q1)*cos(q4) - (4967757600021511*cos(q3)*((4967757600021511*cos(q1)*cos(q2 + pi/2))/81129638414606681695789005144064 - sin(q1)*sin(q2 + pi/2)))/81129638414606681695789005144064 + (4967757600021511*sin(q3)*((4967757600021511*cos(q1)*sin(q2 + pi/2))/81129638414606681695789005144064 + cos(q2 + pi/2)*sin(q1)))/81129638414606681695789005144064 + (4967757600021511*cos(q4)*(cos(q3)*((4967757600021511*cos(q1)*cos(q2 + pi/2))/81129638414606681695789005144064 - sin(q1)*sin(q2 + pi/2)) - sin(q3)*((4967757600021511*cos(q1)*sin(q2 + pi/2))/81129638414606681695789005144064 + cos(q2 + pi/2)*sin(q1))))/81129638414606681695789005144064 - sin(q4)*(cos(q3)*((4967757600021511*cos(q1)*sin(q2 + pi/2))/81129638414606681695789005144064 + cos(q2 + pi/2)*sin(q1)) + sin(q3)*((4967757600021511*cos(q1)*cos(q2 + pi/2))/81129638414606681695789005144064 - sin(q1)*sin(q2 + pi/2)))))/40564819207303340847894502572032;
R(2,3)= (122597380068651197257713859414983140362437055831*cos(q1))/533996758980227520598755426542388028650676130589163192486760401955554931445160137505740521734144 + (4967757600021511*cos(q1)*cos(q4))/81129638414606681695789005144064 - (24678615572571482867467662723121*cos(q3)*((4967757600021511*cos(q1)*cos(q2 + pi/2))/81129638414606681695789005144064 - sin(q1)*sin(q2 + pi/2)))/6582018229284824168619876730229402019930943462534319453394436096 + (24678615572571482867467662723121*sin(q3)*((4967757600021511*cos(q1)*sin(q2 + pi/2))/81129638414606681695789005144064 + cos(q2 + pi/2)*sin(q1)))/6582018229284824168619876730229402019930943462534319453394436096 + cos(q5)*((4967757600021511*cos(q1))/81129638414606681695789005144064 - cos(q3)*((4967757600021511*cos(q1)*cos(q2 + pi/2))/81129638414606681695789005144064 - sin(q1)*sin(q2 + pi/2)) + sin(q3)*((4967757600021511*cos(q1)*sin(q2 + pi/2))/81129638414606681695789005144064 + cos(q2 + pi/2)*sin(q1))) - (4967757600021511*cos(q5)*(cos(q1)*cos(q4) + (4967757600021511*cos(q4)*(cos(q3)*((4967757600021511*cos(q1)*cos(q2 + pi/2))/81129638414606681695789005144064 - sin(q1)*sin(q2 + pi/2)) - sin(q3)*((4967757600021511*cos(q1)*sin(q2 + pi/2))/81129638414606681695789005144064 + cos(q2 + pi/2)*sin(q1))))/81129638414606681695789005144064 - sin(q4)*(cos(q3)*((4967757600021511*cos(q1)*sin(q2 + pi/2))/81129638414606681695789005144064 + cos(q2 + pi/2)*sin(q1)) + sin(q3)*((4967757600021511*cos(q1)*cos(q2 + pi/2))/81129638414606681695789005144064 - sin(q1)*sin(q2 + pi/2)))))/81129638414606681695789005144064 + sin(q5)*(cos(q1)*sin(q4) + cos(q4)*(cos(q3)*((4967757600021511*cos(q1)*sin(q2 + pi/2))/81129638414606681695789005144064 + cos(q2 + pi/2)*sin(q1)) + sin(q3)*((4967757600021511*cos(q1)*cos(q2 + pi/2))/81129638414606681695789005144064 - sin(q1)*sin(q2 + pi/2))) + (4967757600021511*sin(q4)*(cos(q3)*((4967757600021511*cos(q1)*cos(q2 + pi/2))/81129638414606681695789005144064 - sin(q1)*sin(q2 + pi/2)) - sin(q3)*((4967757600021511*cos(q1)*sin(q2 + pi/2))/81129638414606681695789005144064 + cos(q2 + pi/2)*sin(q1))))/81129638414606681695789005144064) + (24678615572571482867467662723121*cos(q4)*(cos(q3)*((4967757600021511*cos(q1)*cos(q2 + pi/2))/81129638414606681695789005144064 - sin(q1)*sin(q2 + pi/2)) - sin(q3)*((4967757600021511*cos(q1)*sin(q2 + pi/2))/81129638414606681695789005144064 + cos(q2 + pi/2)*sin(q1))))/6582018229284824168619876730229402019930943462534319453394436096 - (4967757600021511*sin(q4)*(cos(q3)*((4967757600021511*cos(q1)*sin(q2 + pi/2))/81129638414606681695789005144064 + cos(q2 + pi/2)*sin(q1)) + sin(q3)*((4967757600021511*cos(q1)*cos(q2 + pi/2))/81129638414606681695789005144064 - sin(q1)*sin(q2 + pi/2))))/81129638414606681695789005144064;
R(3,1)= (4967757600021511*sin(q6)*((4967757600021511*cos(q5)*((4967757600021511*cos(q4))/81129638414606681695789005144064 - (4967757600021511*cos(q4)*(cos(q3)*cos(q2 + pi/2) - sin(q3)*sin(q2 + pi/2)))/81129638414606681695789005144064 + sin(q4)*(cos(q3)*sin(q2 + pi/2) + cos(q2 + pi/2)*sin(q3))))/81129638414606681695789005144064 + sin(q5)*(cos(q4)*(cos(q3)*sin(q2 + pi/2) + cos(q2 + pi/2)*sin(q3)) - (4967757600021511*sin(q4))/81129638414606681695789005144064 + (4967757600021511*sin(q4)*(cos(q3)*cos(q2 + pi/2) - sin(q3)*sin(q2 + pi/2)))/81129638414606681695789005144064) - cos(q5)*(cos(q3)*cos(q2 + pi/2) - sin(q3)*sin(q2 + pi/2) + 24678615572571482867467662723121/6582018229284824168619876730229402019930943462534319453394436096)))/81129638414606681695789005144064 - cos(q6)*(cos(q5)*(cos(q4)*(cos(q3)*sin(q2 + pi/2) + cos(q2 + pi/2)*sin(q3)) - (4967757600021511*sin(q4))/81129638414606681695789005144064 + (4967757600021511*sin(q4)*(cos(q3)*cos(q2 + pi/2) - sin(q3)*sin(q2 + pi/2)))/81129638414606681695789005144064) - (4967757600021511*sin(q5)*((4967757600021511*cos(q4))/81129638414606681695789005144064 - (4967757600021511*cos(q4)*(cos(q3)*cos(q2 + pi/2) - sin(q3)*sin(q2 + pi/2)))/81129638414606681695789005144064 + sin(q4)*(cos(q3)*sin(q2 + pi/2) + cos(q2 + pi/2)*sin(q3))))/81129638414606681695789005144064 + sin(q5)*(cos(q3)*cos(q2 + pi/2) - sin(q3)*sin(q2 + pi/2) + 24678615572571482867467662723121/6582018229284824168619876730229402019930943462534319453394436096)) - (24678615572571482867467662723121*cos(q6)*((4967757600021511*cos(q5)*((4967757600021511*cos(q4))/81129638414606681695789005144064 - (4967757600021511*cos(q4)*(cos(q3)*cos(q2 + pi/2) - sin(q3)*sin(q2 + pi/2)))/81129638414606681695789005144064 + sin(q4)*(cos(q3)*sin(q2 + pi/2) + cos(q2 + pi/2)*sin(q3))))/81129638414606681695789005144064 + sin(q5)*(cos(q4)*(cos(q3)*sin(q2 + pi/2) + cos(q2 + pi/2)*sin(q3)) - (4967757600021511*sin(q4))/81129638414606681695789005144064 + (4967757600021511*sin(q4)*(cos(q3)*cos(q2 + pi/2) - sin(q3)*sin(q2 + pi/2)))/81129638414606681695789005144064) - cos(q5)*(cos(q3)*cos(q2 + pi/2) - sin(q3)*sin(q2 + pi/2) + 24678615572571482867467662723121/6582018229284824168619876730229402019930943462534319453394436096)))/3291009114642412084309938365114701009965471731267159726697218048 - (4967757600021511*sin(q6)*(cos(q5)*(cos(q4)*(cos(q3)*sin(q2 + pi/2) + cos(q2 + pi/2)*sin(q3)) - (4967757600021511*sin(q4))/81129638414606681695789005144064 + (4967757600021511*sin(q4)*(cos(q3)*cos(q2 + pi/2) - sin(q3)*sin(q2 + pi/2)))/81129638414606681695789005144064) - (4967757600021511*sin(q5)*((4967757600021511*cos(q4))/81129638414606681695789005144064 - (4967757600021511*cos(q4)*(cos(q3)*cos(q2 + pi/2) - sin(q3)*sin(q2 + pi/2)))/81129638414606681695789005144064 + sin(q4)*(cos(q3)*sin(q2 + pi/2) + cos(q2 + pi/2)*sin(q3))))/81129638414606681695789005144064 + sin(q5)*(cos(q3)*cos(q2 + pi/2) - sin(q3)*sin(q2 + pi/2) + 24678615572571482867467662723121/6582018229284824168619876730229402019930943462534319453394436096)))/40564819207303340847894502572032 - (4967757600021511*cos(q6)*((4967757600021511*cos(q4))/81129638414606681695789005144064 + (4967757600021511*cos(q3)*cos(q2 + pi/2))/81129638414606681695789005144064 - (4967757600021511*sin(q3)*sin(q2 + pi/2))/81129638414606681695789005144064 - (4967757600021511*cos(q4)*(cos(q3)*cos(q2 + pi/2) - sin(q3)*sin(q2 + pi/2)))/81129638414606681695789005144064 + sin(q4)*(cos(q3)*sin(q2 + pi/2) + cos(q2 + pi/2)*sin(q3)) + 122597380068651197257713859414983140362437055831/533996758980227520598755426542388028650676130589163192486760401955554931445160137505740521734144))/40564819207303340847894502572032 + sin(q6)*((4967757600021511*cos(q4))/81129638414606681695789005144064 + (4967757600021511*cos(q3)*cos(q2 + pi/2))/81129638414606681695789005144064 - (4967757600021511*sin(q3)*sin(q2 + pi/2))/81129638414606681695789005144064 - (4967757600021511*cos(q4)*(cos(q3)*cos(q2 + pi/2) - sin(q3)*sin(q2 + pi/2)))/81129638414606681695789005144064 + sin(q4)*(cos(q3)*sin(q2 + pi/2) + cos(q2 + pi/2)*sin(q3)) + 122597380068651197257713859414983140362437055831/533996758980227520598755426542388028650676130589163192486760401955554931445160137505740521734144); 
R(3,2)= (4967757600021511*cos(q6)*((4967757600021511*cos(q5)*((4967757600021511*cos(q4))/81129638414606681695789005144064 - (4967757600021511*cos(q4)*(cos(q3)*cos(q2 + pi/2) - sin(q3)*sin(q2 + pi/2)))/81129638414606681695789005144064 + sin(q4)*(cos(q3)*sin(q2 + pi/2) + cos(q2 + pi/2)*sin(q3))))/81129638414606681695789005144064 + sin(q5)*(cos(q4)*(cos(q3)*sin(q2 + pi/2) + cos(q2 + pi/2)*sin(q3)) - (4967757600021511*sin(q4))/81129638414606681695789005144064 + (4967757600021511*sin(q4)*(cos(q3)*cos(q2 + pi/2) - sin(q3)*sin(q2 + pi/2)))/81129638414606681695789005144064) - cos(q5)*(cos(q3)*cos(q2 + pi/2) - sin(q3)*sin(q2 + pi/2) + 24678615572571482867467662723121/6582018229284824168619876730229402019930943462534319453394436096)))/81129638414606681695789005144064 - (4967757600021511*cos(q6)*(cos(q5)*(cos(q4)*(cos(q3)*sin(q2 + pi/2) + cos(q2 + pi/2)*sin(q3)) - (4967757600021511*sin(q4))/81129638414606681695789005144064 + (4967757600021511*sin(q4)*(cos(q3)*cos(q2 + pi/2) - sin(q3)*sin(q2 + pi/2)))/81129638414606681695789005144064) - (4967757600021511*sin(q5)*((4967757600021511*cos(q4))/81129638414606681695789005144064 - (4967757600021511*cos(q4)*(cos(q3)*cos(q2 + pi/2) - sin(q3)*sin(q2 + pi/2)))/81129638414606681695789005144064 + sin(q4)*(cos(q3)*sin(q2 + pi/2) + cos(q2 + pi/2)*sin(q3))))/81129638414606681695789005144064 + sin(q5)*(cos(q3)*cos(q2 + pi/2) - sin(q3)*sin(q2 + pi/2) + 24678615572571482867467662723121/6582018229284824168619876730229402019930943462534319453394436096)))/40564819207303340847894502572032 + (24678615572571482867467662723121*sin(q6)*((4967757600021511*cos(q5)*((4967757600021511*cos(q4))/81129638414606681695789005144064 - (4967757600021511*cos(q4)*(cos(q3)*cos(q2 + pi/2) - sin(q3)*sin(q2 + pi/2)))/81129638414606681695789005144064 + sin(q4)*(cos(q3)*sin(q2 + pi/2) + cos(q2 + pi/2)*sin(q3))))/81129638414606681695789005144064 + sin(q5)*(cos(q4)*(cos(q3)*sin(q2 + pi/2) + cos(q2 + pi/2)*sin(q3)) - (4967757600021511*sin(q4))/81129638414606681695789005144064 + (4967757600021511*sin(q4)*(cos(q3)*cos(q2 + pi/2) - sin(q3)*sin(q2 + pi/2)))/81129638414606681695789005144064) - cos(q5)*(cos(q3)*cos(q2 + pi/2) - sin(q3)*sin(q2 + pi/2) + 24678615572571482867467662723121/6582018229284824168619876730229402019930943462534319453394436096)))/3291009114642412084309938365114701009965471731267159726697218048 + sin(q6)*(cos(q5)*(cos(q4)*(cos(q3)*sin(q2 + pi/2) + cos(q2 + pi/2)*sin(q3)) - (4967757600021511*sin(q4))/81129638414606681695789005144064 + (4967757600021511*sin(q4)*(cos(q3)*cos(q2 + pi/2) - sin(q3)*sin(q2 + pi/2)))/81129638414606681695789005144064) - (4967757600021511*sin(q5)*((4967757600021511*cos(q4))/81129638414606681695789005144064 - (4967757600021511*cos(q4)*(cos(q3)*cos(q2 + pi/2) - sin(q3)*sin(q2 + pi/2)))/81129638414606681695789005144064 + sin(q4)*(cos(q3)*sin(q2 + pi/2) + cos(q2 + pi/2)*sin(q3))))/81129638414606681695789005144064 + sin(q5)*(cos(q3)*cos(q2 + pi/2) - sin(q3)*sin(q2 + pi/2) + 24678615572571482867467662723121/6582018229284824168619876730229402019930943462534319453394436096)) + cos(q6)*((4967757600021511*cos(q4))/81129638414606681695789005144064 + (4967757600021511*cos(q3)*cos(q2 + pi/2))/81129638414606681695789005144064 - (4967757600021511*sin(q3)*sin(q2 + pi/2))/81129638414606681695789005144064 - (4967757600021511*cos(q4)*(cos(q3)*cos(q2 + pi/2) - sin(q3)*sin(q2 + pi/2)))/81129638414606681695789005144064 + sin(q4)*(cos(q3)*sin(q2 + pi/2) + cos(q2 + pi/2)*sin(q3)) + 122597380068651197257713859414983140362437055831/533996758980227520598755426542388028650676130589163192486760401955554931445160137505740521734144) + (4967757600021511*sin(q6)*((4967757600021511*cos(q4))/81129638414606681695789005144064 + (4967757600021511*cos(q3)*cos(q2 + pi/2))/81129638414606681695789005144064 - (4967757600021511*sin(q3)*sin(q2 + pi/2))/81129638414606681695789005144064 - (4967757600021511*cos(q4)*(cos(q3)*cos(q2 + pi/2) - sin(q3)*sin(q2 + pi/2)))/81129638414606681695789005144064 + sin(q4)*(cos(q3)*sin(q2 + pi/2) + cos(q2 + pi/2)*sin(q3)) + 122597380068651197257713859414983140362437055831/533996758980227520598755426542388028650676130589163192486760401955554931445160137505740521734144))/40564819207303340847894502572032;
R(3,3)=  (24678615572571482867467662723121*cos(q4))/6582018229284824168619876730229402019930943462534319453394436096 - (4967757600021511*cos(q5)*((4967757600021511*cos(q4))/81129638414606681695789005144064 - (4967757600021511*cos(q4)*(cos(q3)*cos(q2 + pi/2) - sin(q3)*sin(q2 + pi/2)))/81129638414606681695789005144064 + sin(q4)*(cos(q3)*sin(q2 + pi/2) + cos(q2 + pi/2)*sin(q3))))/81129638414606681695789005144064 + (24678615572571482867467662723121*cos(q3)*cos(q2 + pi/2))/6582018229284824168619876730229402019930943462534319453394436096 - sin(q5)*(cos(q4)*(cos(q3)*sin(q2 + pi/2) + cos(q2 + pi/2)*sin(q3)) - (4967757600021511*sin(q4))/81129638414606681695789005144064 + (4967757600021511*sin(q4)*(cos(q3)*cos(q2 + pi/2) - sin(q3)*sin(q2 + pi/2)))/81129638414606681695789005144064) + cos(q5)*(cos(q3)*cos(q2 + pi/2) - sin(q3)*sin(q2 + pi/2) + 24678615572571482867467662723121/6582018229284824168619876730229402019930943462534319453394436096) - (24678615572571482867467662723121*sin(q3)*sin(q2 + pi/2))/6582018229284824168619876730229402019930943462534319453394436096 - (24678615572571482867467662723121*cos(q4)*(cos(q3)*cos(q2 + pi/2) - sin(q3)*sin(q2 + pi/2)))/6582018229284824168619876730229402019930943462534319453394436096 + (4967757600021511*sin(q4)*(cos(q3)*sin(q2 + pi/2) + cos(q2 + pi/2)*sin(q3)))/81129638414606681695789005144064 + 609034066578767699168763939638324732237239140958410949107980641/43322963970637732180912721627235682866194329302747133987038743447103457934462900359999600095377180907771737671271930809827721216;

x= (3093548567763867359251342063207821441907716257110899757329320000341*cos(q3)*(cos(q1)*sin(q2 + pi/2) + (4967757600021511*cos(q2 + pi/2)*sin(q1))/81129638414606681695789005144064))/6582018229284824168619876730229402019930943462534319453394436096000 - (11*cos(q3)*(cos(q1)*cos(q2 + pi/2) - (4967757600021511*sin(q1)*sin(q2 + pi/2))/81129638414606681695789005144064))/100 - (15367999408544611283610854417045082301222635242944759808457209068371609267073198931*sin(q1))/533996758980227520598755426542388028650676130589163192486760401955554931445160137505740521734144000 - (111*cos(q1)*cos(q2 + pi/2))/250 - (501743517602172611*cos(q4)*sin(q1))/81129638414606681695789005144064000 + (3093548567763867359251342063207821441907716257110899757329320000341*sin(q3)*(cos(q1)*cos(q2 + pi/2) - (4967757600021511*sin(q1)*sin(q2 + pi/2))/81129638414606681695789005144064))/6582018229284824168619876730229402019930943462534319453394436096000 + (11*sin(q3)*(cos(q1)*sin(q2 + pi/2) + (4967757600021511*cos(q2 + pi/2)*sin(q1))/81129638414606681695789005144064))/100 + (551421093602387721*sin(q1)*sin(q2 + pi/2))/20282409603651670423947251286016000 + (101*cos(q5)*(cos(q3)*(cos(q1)*sin(q2 + pi/2) + (4967757600021511*cos(q2 + pi/2)*sin(q1))/81129638414606681695789005144064) - (4967757600021511*sin(q1))/81129638414606681695789005144064 + sin(q3)*(cos(q1)*cos(q2 + pi/2) - (4967757600021511*sin(q1)*sin(q2 + pi/2))/81129638414606681695789005144064)))/1000 + (2*sin(q5)*(cos(q3)*(cos(q1)*sin(q2 + pi/2) + (4967757600021511*cos(q2 + pi/2)*sin(q1))/81129638414606681695789005144064) - (4967757600021511*sin(q1))/81129638414606681695789005144064 + sin(q3)*(cos(q1)*cos(q2 + pi/2) - (4967757600021511*sin(q1)*sin(q2 + pi/2))/81129638414606681695789005144064)))/25 + (501743517602172611*cos(q5)*(cos(q4)*sin(q1) + (4967757600021511*cos(q4)*(cos(q3)*(cos(q1)*sin(q2 + pi/2) + (4967757600021511*cos(q2 + pi/2)*sin(q1))/81129638414606681695789005144064) + sin(q3)*(cos(q1)*cos(q2 + pi/2) - (4967757600021511*sin(q1)*sin(q2 + pi/2))/81129638414606681695789005144064)))/81129638414606681695789005144064 + sin(q4)*(cos(q3)*(cos(q1)*cos(q2 + pi/2) - (4967757600021511*sin(q1)*sin(q2 + pi/2))/81129638414606681695789005144064) - sin(q3)*(cos(q1)*sin(q2 + pi/2) + (4967757600021511*cos(q2 + pi/2)*sin(q1))/81129638414606681695789005144064))))/81129638414606681695789005144064000 + (4967757600021511*sin(q5)*(cos(q4)*sin(q1) + (4967757600021511*cos(q4)*(cos(q3)*(cos(q1)*sin(q2 + pi/2) + (4967757600021511*cos(q2 + pi/2)*sin(q1))/81129638414606681695789005144064) + sin(q3)*(cos(q1)*cos(q2 + pi/2) - (4967757600021511*sin(q1)*sin(q2 + pi/2))/81129638414606681695789005144064)))/81129638414606681695789005144064 + sin(q4)*(cos(q3)*(cos(q1)*cos(q2 + pi/2) - (4967757600021511*sin(q1)*sin(q2 + pi/2))/81129638414606681695789005144064) - sin(q3)*(cos(q1)*sin(q2 + pi/2) + (4967757600021511*cos(q2 + pi/2)*sin(q1))/81129638414606681695789005144064))))/1014120480182583521197362564300800 + (2*cos(q5)*(sin(q1)*sin(q4) - cos(q4)*(cos(q3)*(cos(q1)*cos(q2 + pi/2) - (4967757600021511*sin(q1)*sin(q2 + pi/2))/81129638414606681695789005144064) - sin(q3)*(cos(q1)*sin(q2 + pi/2) + (4967757600021511*cos(q2 + pi/2)*sin(q1))/81129638414606681695789005144064)) + (4967757600021511*sin(q4)*(cos(q3)*(cos(q1)*sin(q2 + pi/2) + (4967757600021511*cos(q2 + pi/2)*sin(q1))/81129638414606681695789005144064) + sin(q3)*(cos(q1)*cos(q2 + pi/2) - (4967757600021511*sin(q1)*sin(q2 + pi/2))/81129638414606681695789005144064)))/81129638414606681695789005144064))/25 - (101*sin(q5)*(sin(q1)*sin(q4) - cos(q4)*(cos(q3)*(cos(q1)*cos(q2 + pi/2) - (4967757600021511*sin(q1)*sin(q2 + pi/2))/81129638414606681695789005144064) - sin(q3)*(cos(q1)*sin(q2 + pi/2) + (4967757600021511*cos(q2 + pi/2)*sin(q1))/81129638414606681695789005144064)) + (4967757600021511*sin(q4)*(cos(q3)*(cos(q1)*sin(q2 + pi/2) + (4967757600021511*cos(q2 + pi/2)*sin(q1))/81129638414606681695789005144064) + sin(q3)*(cos(q1)*cos(q2 + pi/2) - (4967757600021511*sin(q1)*sin(q2 + pi/2))/81129638414606681695789005144064)))/81129638414606681695789005144064))/1000 - (2492540172829719769614233935035221*cos(q4)*(cos(q3)*(cos(q1)*sin(q2 + pi/2) + (4967757600021511*cos(q2 + pi/2)*sin(q1))/81129638414606681695789005144064) + sin(q3)*(cos(q1)*cos(q2 + pi/2) - (4967757600021511*sin(q1)*sin(q2 + pi/2))/81129638414606681695789005144064)))/6582018229284824168619876730229402019930943462534319453394436096000 - (501743517602172611*sin(q4)*(cos(q3)*(cos(q1)*cos(q2 + pi/2) - (4967757600021511*sin(q1)*sin(q2 + pi/2))/81129638414606681695789005144064) - sin(q3)*(cos(q1)*sin(q2 + pi/2) + (4967757600021511*cos(q2 + pi/2)*sin(q1))/81129638414606681695789005144064)))/81129638414606681695789005144064000;
y= (15367999408544611283610854417045082301222635242944759808457209068371609267073198931*cos(q1))/533996758980227520598755426542388028650676130589163192486760401955554931445160137505740521734144000 + (501743517602172611*cos(q1)*cos(q4))/81129638414606681695789005144064000 - (11*cos(q3)*((4967757600021511*cos(q1)*sin(q2 + pi/2))/81129638414606681695789005144064 + cos(q2 + pi/2)*sin(q1)))/100 - (3093548567763867359251342063207821441907716257110899757329320000341*cos(q3)*((4967757600021511*cos(q1)*cos(q2 + pi/2))/81129638414606681695789005144064 - sin(q1)*sin(q2 + pi/2)))/6582018229284824168619876730229402019930943462534319453394436096000 + (3093548567763867359251342063207821441907716257110899757329320000341*sin(q3)*((4967757600021511*cos(q1)*sin(q2 + pi/2))/81129638414606681695789005144064 + cos(q2 + pi/2)*sin(q1)))/6582018229284824168619876730229402019930943462534319453394436096000 - (11*sin(q3)*((4967757600021511*cos(q1)*cos(q2 + pi/2))/81129638414606681695789005144064 - sin(q1)*sin(q2 + pi/2)))/100 - (551421093602387721*cos(q1)*sin(q2 + pi/2))/20282409603651670423947251286016000 - (111*cos(q2 + pi/2)*sin(q1))/250 + (101*cos(q5)*((4967757600021511*cos(q1))/81129638414606681695789005144064 - cos(q3)*((4967757600021511*cos(q1)*cos(q2 + pi/2))/81129638414606681695789005144064 - sin(q1)*sin(q2 + pi/2)) + sin(q3)*((4967757600021511*cos(q1)*sin(q2 + pi/2))/81129638414606681695789005144064 + cos(q2 + pi/2)*sin(q1))))/1000 + (2*sin(q5)*((4967757600021511*cos(q1))/81129638414606681695789005144064 - cos(q3)*((4967757600021511*cos(q1)*cos(q2 + pi/2))/81129638414606681695789005144064 - sin(q1)*sin(q2 + pi/2)) + sin(q3)*((4967757600021511*cos(q1)*sin(q2 + pi/2))/81129638414606681695789005144064 + cos(q2 + pi/2)*sin(q1))))/25 - (501743517602172611*cos(q5)*(cos(q1)*cos(q4) + (4967757600021511*cos(q4)*(cos(q3)*((4967757600021511*cos(q1)*cos(q2 + pi/2))/81129638414606681695789005144064 - sin(q1)*sin(q2 + pi/2)) - sin(q3)*((4967757600021511*cos(q1)*sin(q2 + pi/2))/81129638414606681695789005144064 + cos(q2 + pi/2)*sin(q1))))/81129638414606681695789005144064 - sin(q4)*(cos(q3)*((4967757600021511*cos(q1)*sin(q2 + pi/2))/81129638414606681695789005144064 + cos(q2 + pi/2)*sin(q1)) + sin(q3)*((4967757600021511*cos(q1)*cos(q2 + pi/2))/81129638414606681695789005144064 - sin(q1)*sin(q2 + pi/2)))))/81129638414606681695789005144064000 - (2*cos(q5)*(cos(q1)*sin(q4) + cos(q4)*(cos(q3)*((4967757600021511*cos(q1)*sin(q2 + pi/2))/81129638414606681695789005144064 + cos(q2 + pi/2)*sin(q1)) + sin(q3)*((4967757600021511*cos(q1)*cos(q2 + pi/2))/81129638414606681695789005144064 - sin(q1)*sin(q2 + pi/2))) + (4967757600021511*sin(q4)*(cos(q3)*((4967757600021511*cos(q1)*cos(q2 + pi/2))/81129638414606681695789005144064 - sin(q1)*sin(q2 + pi/2)) - sin(q3)*((4967757600021511*cos(q1)*sin(q2 + pi/2))/81129638414606681695789005144064 + cos(q2 + pi/2)*sin(q1))))/81129638414606681695789005144064))/25 - (4967757600021511*sin(q5)*(cos(q1)*cos(q4) + (4967757600021511*cos(q4)*(cos(q3)*((4967757600021511*cos(q1)*cos(q2 + pi/2))/81129638414606681695789005144064 - sin(q1)*sin(q2 + pi/2)) - sin(q3)*((4967757600021511*cos(q1)*sin(q2 + pi/2))/81129638414606681695789005144064 + cos(q2 + pi/2)*sin(q1))))/81129638414606681695789005144064 - sin(q4)*(cos(q3)*((4967757600021511*cos(q1)*sin(q2 + pi/2))/81129638414606681695789005144064 + cos(q2 + pi/2)*sin(q1)) + sin(q3)*((4967757600021511*cos(q1)*cos(q2 + pi/2))/81129638414606681695789005144064 - sin(q1)*sin(q2 + pi/2)))))/1014120480182583521197362564300800 + (101*sin(q5)*(cos(q1)*sin(q4) + cos(q4)*(cos(q3)*((4967757600021511*cos(q1)*sin(q2 + pi/2))/81129638414606681695789005144064 + cos(q2 + pi/2)*sin(q1)) + sin(q3)*((4967757600021511*cos(q1)*cos(q2 + pi/2))/81129638414606681695789005144064 - sin(q1)*sin(q2 + pi/2))) + (4967757600021511*sin(q4)*(cos(q3)*((4967757600021511*cos(q1)*cos(q2 + pi/2))/81129638414606681695789005144064 - sin(q1)*sin(q2 + pi/2)) - sin(q3)*((4967757600021511*cos(q1)*sin(q2 + pi/2))/81129638414606681695789005144064 + cos(q2 + pi/2)*sin(q1))))/81129638414606681695789005144064))/1000 + (2492540172829719769614233935035221*cos(q4)*(cos(q3)*((4967757600021511*cos(q1)*cos(q2 + pi/2))/81129638414606681695789005144064 - sin(q1)*sin(q2 + pi/2)) - sin(q3)*((4967757600021511*cos(q1)*sin(q2 + pi/2))/81129638414606681695789005144064 + cos(q2 + pi/2)*sin(q1))))/6582018229284824168619876730229402019930943462534319453394436096000 - (501743517602172611*sin(q4)*(cos(q3)*((4967757600021511*cos(q1)*sin(q2 + pi/2))/81129638414606681695789005144064 + cos(q2 + pi/2)*sin(q1)) + sin(q3)*((4967757600021511*cos(q1)*cos(q2 + pi/2))/81129638414606681695789005144064 - sin(q1)*sin(q2 + pi/2))))/81129638414606681695789005144064000;
z=  (2492540172829719769614233935035221*cos(q4))/6582018229284824168619876730229402019930943462534319453394436096000 + (111*sin(q2 + pi/2))/250 - (501743517602172611*cos(q5)*((4967757600021511*cos(q4))/81129638414606681695789005144064 - (4967757600021511*cos(q4)*(cos(q3)*cos(q2 + pi/2) - sin(q3)*sin(q2 + pi/2)))/81129638414606681695789005144064 + sin(q4)*(cos(q3)*sin(q2 + pi/2) + cos(q2 + pi/2)*sin(q3))))/81129638414606681695789005144064000 + (2*cos(q5)*(cos(q4)*(cos(q3)*sin(q2 + pi/2) + cos(q2 + pi/2)*sin(q3)) - (4967757600021511*sin(q4))/81129638414606681695789005144064 + (4967757600021511*sin(q4)*(cos(q3)*cos(q2 + pi/2) - sin(q3)*sin(q2 + pi/2)))/81129638414606681695789005144064))/25 - (4967757600021511*sin(q5)*((4967757600021511*cos(q4))/81129638414606681695789005144064 - (4967757600021511*cos(q4)*(cos(q3)*cos(q2 + pi/2) - sin(q3)*sin(q2 + pi/2)))/81129638414606681695789005144064 + sin(q4)*(cos(q3)*sin(q2 + pi/2) + cos(q2 + pi/2)*sin(q3))))/1014120480182583521197362564300800 + (3093548567763867359251342063207821441907716257110899757329320000341*cos(q3)*cos(q2 + pi/2))/6582018229284824168619876730229402019930943462534319453394436096000 - (101*sin(q5)*(cos(q4)*(cos(q3)*sin(q2 + pi/2) + cos(q2 + pi/2)*sin(q3)) - (4967757600021511*sin(q4))/81129638414606681695789005144064 + (4967757600021511*sin(q4)*(cos(q3)*cos(q2 + pi/2) - sin(q3)*sin(q2 + pi/2)))/81129638414606681695789005144064))/1000 + (11*cos(q3)*sin(q2 + pi/2))/100 + (11*cos(q2 + pi/2)*sin(q3))/100 + (101*cos(q5)*(cos(q3)*cos(q2 + pi/2) - sin(q3)*sin(q2 + pi/2) + 24678615572571482867467662723121/6582018229284824168619876730229402019930943462534319453394436096))/1000 - (3093548567763867359251342063207821441907716257110899757329320000341*sin(q3)*sin(q2 + pi/2))/6582018229284824168619876730229402019930943462534319453394436096000 + (2*sin(q5)*(cos(q3)*cos(q2 + pi/2) - sin(q3)*sin(q2 + pi/2) + 24678615572571482867467662723121/6582018229284824168619876730229402019930943462534319453394436096))/25 - (2492540172829719769614233935035221*cos(q4)*(cos(q3)*cos(q2 + pi/2) - sin(q3)*sin(q2 + pi/2)))/6582018229284824168619876730229402019930943462534319453394436096000 + (501743517602172611*sin(q4)*(cos(q3)*sin(q2 + pi/2) + cos(q2 + pi/2)*sin(q3)))/81129638414606681695789005144064000 + 11480585452218999027941871231217532304037356188806668987345873104512650241924954143676919374104305372264095485942494395741528326981/43322963970637732180912721627235682866194329302747133987038743447103457934462900359999600095377180907771737671271930809827721216000;
end
